simulink model "asbCubeSatVehiclePlant"  (R2025b)
settings: Solver=ode23t  StartTime=0.0  StopTime=86400  FixedStep=CubeSatTimeStep  RelTol=1e-5  AbsTol=1e-5  EnableMultiTasking=on
undefined symbols (not defined in the file): CubeSatTimeStep
libraries: asbCubeSatActuatorsLib x1, asbCubeSatSensorsLib x1, asbCubeSatDynamicsLib x1
settings Model: DataDictionary=asbCubeSatArchInterfaceData.sldd  Creator=The MathWorks, Inc.  LastModifiedBy=The MathWorks, Inc.
settings SolverCC: AlgebraicLoopSolver=TrustRegion  MaxZcPerStep=1.0
settings DataIOCC: SaveOutput=off  DSMLogging=off  SaveTime=off
settings DebuggingCC: MergeDetectMultiDrivingBlocksExec=none  UnconnectedLineMsg=warning
settings ModelReferenceCC: EnableRefExpFcnMdlSchedulingChecks=on  ModelReferenceNumInstancesAllowed=Single  PropagateSignalLabelsOutOfModel=off
settings RTWCC: GPUComputeCapability=3.5  DLArmComputeVersion=19.05
settings GRTTargetCC: SubcomponentCodeInterfacePackaging=Nonreusable function

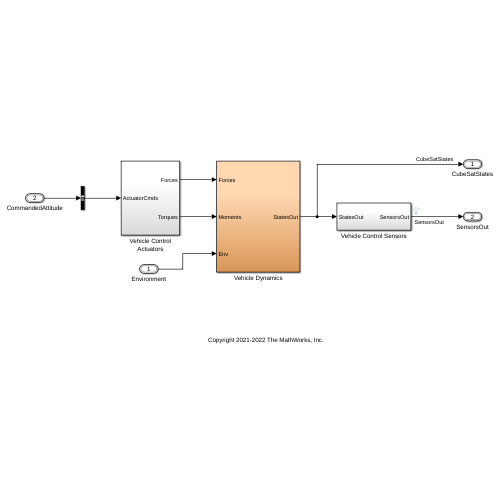
[thumbnail: Simulink's stored preview of the top-level diagram]
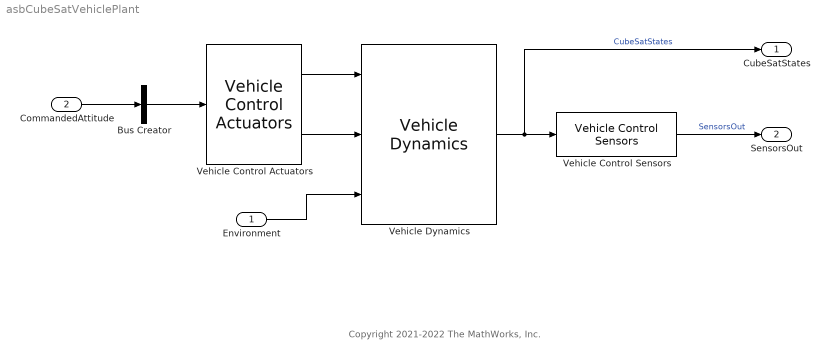
== system asbCubeSatVehiclePlant ==
  note: Copyright 2021-2022 The MathWorks, Inc.
  Environment : Inport  OutDataTypeStr=Bus: EnvBus
  CommandedAttitude : Inport  Port=2  OutDataTypeStr=Bus: ACSOutBus
  Bus Creator : BusCreator  Inputs=1  OutDataTypeStr=Bus: FCSOutBus
      settings: InheritFromInputs=off
  Vehicle Control Actuators : asbCubeSatActuatorsLib/Vehicle Control Actuators  SystemSampleTime=-1  VariantActivationTime=update diagram  EmptyChoice=off  PassThrough=off  PassThroughVariantControl=(default)  EmptyChoiceVariantControl=(default)  AllowFlexibleInterface=on  Latency=0  AutoFrameSizeCalculation=off
  Vehicle Control Sensors : asbCubeSatSensorsLib/Vehicle Control Sensors  SystemSampleTime=-1  VariantActivationTime=update diagram  EmptyChoice=off  PassThrough=off  PassThroughVariantControl=(default)  EmptyChoiceVariantControl=(default)  AllowFlexibleInterface=on  Latency=0  AutoFrameSizeCalculation=off
  Vehicle Dynamics : asbCubeSatDynamicsLib/Vehicle Dynamics  SystemSampleTime=-1  VariantActivationTime=update diagram  EmptyChoice=off  PassThrough=off  PassThroughVariantControl=(default)  EmptyChoiceVariantControl=(default)  AllowFlexibleInterface=on  Latency=0  AutoFrameSizeCalculation=off
  CubeSatStates : Outport  OutDataTypeStr=Bus: StatesOutBus  SampleTime=0
  SensorsOut : Outport  Port=2  OutDataTypeStr=Bus: StatesOutBus  SampleTime=CubeSatTimeStep  BusOutputAsStruct=on
  wires:
  Vehicle Control Sensors/1 -> SensorsOut/1  "SensorsOut"
  CommandedAttitude/1 -> Bus Creator/1
  Vehicle Control Actuators/2 -> Vehicle Dynamics/2
  Vehicle Control Actuators/1 -> Vehicle Dynamics/1
  Vehicle Dynamics/1 -> Vehicle Control Sensors/1, CubeSatStates/1  "CubeSatStates"
  Environment/1 -> Vehicle Dynamics/3
  Bus Creator/1 -> Vehicle Control Actuators/1
